simulink model "mte484lab3partc2"  (R2024a)
settings: Solver=VariableStepAuto  StartTime=0.0  StopTime=60.0  MaxStep=0.001  RelTol=1e-3
values from neighbouring files (symbols this model uses):
  C2den = [1 Pd(2) 0]    [mte484lab3partcsetup.m]
  C2num = [-7 -2.45]    [mte484lab3partasetup.m]    (also in mte484lab3partcsetup.m = -Pd(3:5)/g)
  Cden = [1 pc]    [mte484lab3partcsetup.m]
  Cnum = -k*[1 zc]    [mte484lab3partcsetup.m]
  K1 = -1.883    [mte484lab3partcsetup.m]
  K2 = 0.0609    [mte484lab3parta.m]    (also in mte484lab3partasetup.m; mte484lab3partcsetup.m)
  K3 = -4.526    [mte484lab3parta.m]    (also in mte484lab3partasetup.m; mte484lab3partcsetup.m)
  sat = 0.7    [mte484lab3parta.m]    (also in mte484lab3partasetup.m; mte484lab3partcsetup.m)
  tau = 0.0216    [mte484lab3partcsetup.m]
  Ts = 0.001    [mte484lab3parta.m]    (also in mte484lab3partasetup.m; mte484lab3partbsetup.m; mte484lab3partcsetup.m)
undefined symbols (not defined in the file or in its folder): D2den, D2num, Dden, Dnum
settings Model: Creator=christopherkoo  LastModifiedBy=christopherkoo

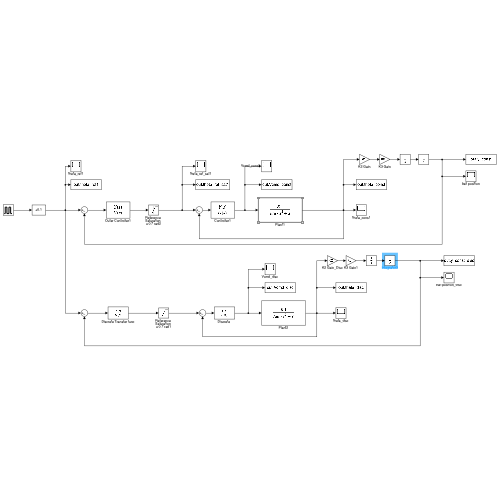
[thumbnail: Simulink's stored preview of the top-level diagram]
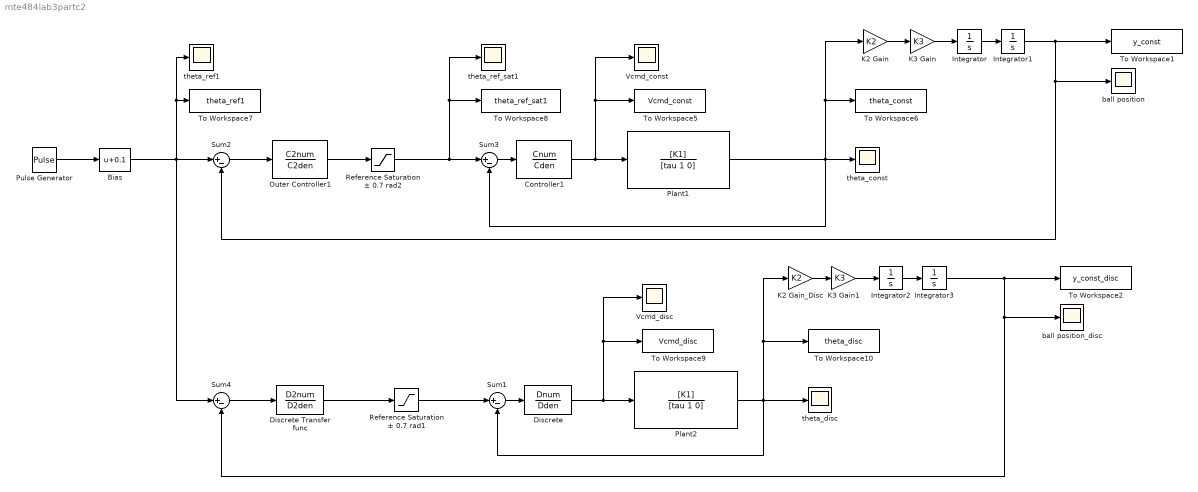
== system mte484lab3partc2 ==
  Bias : Bias  Bias=0.1  SaturateOnIntegerOverflow=off
  Controller1 : TransferFcn  Numerator=Cnum  Denominator=Cden
  "Discrete " : DiscreteTransferFcn  Numerator=Dnum  Denominator=Dden  SampleTime=Ts
  Discrete Transfer func : DiscreteTransferFcn  Numerator=D2num  Denominator=D2den  SampleTime=Ts
  Integrator : Integrator
  Integrator1 : Integrator  InitialCondition=0.1
  Integrator2 : Integrator
  Integrator3 : Integrator  InitialCondition=0.1
  K2 Gain : Gain  Gain=K2
  K2 Gain_Disc : Gain  Gain=K2
  K3 Gain : Gain  Gain=K3
  K3 Gain1 : Gain  Gain=K3
  Outer Controller1 : TransferFcn  Numerator=C2num  Denominator=C2den
  Plant1 : TransferFcn  Numerator=[K1]  Denominator=[tau 1 0]
  Plant2 : TransferFcn  Numerator=[K1]  Denominator=[tau 1 0]
  Pulse Generator : DiscretePulseGenerator  PulseType=Time based  Amplitude=0.15  Period=20  PulseWidth=50
  Reference Saturation ± 0.7 rad1 : Saturate  UpperLimit=sat  LowerLimit=-sat
  Reference Saturation ± 0.7 rad2 : Saturate  UpperLimit=sat  LowerLimit=-sat
  Sum{1..4} (4 alike) : Sum  Inputs=|+-
  To Workspace1 : ToWorkspace  VariableName=y_const  SaveFormat=Timeseries  SampleTime=-1
  To Workspace10 : ToWorkspace  VariableName=theta_disc  SaveFormat=Timeseries  SampleTime=-1
  To Workspace2 : ToWorkspace  VariableName=y_const_disc  SaveFormat=Timeseries  SampleTime=-1
  To Workspace5 : ToWorkspace  VariableName=Vcmd_const  SaveFormat=Timeseries  SampleTime=-1
  To Workspace6 : ToWorkspace  VariableName=theta_const  SaveFormat=Timeseries  SampleTime=-1
  To Workspace7 : ToWorkspace  VariableName=theta_ref1  SaveFormat=Timeseries  SampleTime=-1
  To Workspace8 : ToWorkspace  VariableName=theta_ref_sat1  SaveFormat=Timeseries  SampleTime=-1
  To Workspace9 : ToWorkspace  VariableName=Vcmd_disc  SaveFormat=Timeseries  SampleTime=-1
  Vcmd_const : Scope
  Vcmd_disc : Scope
  ball position : Scope
  ball position_disc : Scope
  theta_const : Scope
  theta_disc : Scope
  theta_ref1 : Scope
  theta_ref_sat1 : Scope
  wires:
  Bias/1 -> Sum4/1, Sum2/1, theta_ref1/1, To Workspace7/1
  Controller1/1 -> Plant1/1, Vcmd_const/1, To Workspace5/1
  Sum1/1 -> "Discrete "/1
  Sum3/1 -> Controller1/1
  Plant2/1 -> K2 Gain_Disc/1, To Workspace10/1, theta_disc/1, Sum1/2
  "Discrete "/1 -> Plant2/1, Vcmd_disc/1, To Workspace9/1
  Reference Saturation ± 0.7 rad2/1 -> To Workspace8/1, theta_ref_sat1/1, Sum3/1
  Outer Controller1/1 -> Reference Saturation ± 0.7 rad2/1
  Sum2/1 -> Outer Controller1/1
  Plant1/1 -> Sum3/2, K2 Gain/1, To Workspace6/1, theta_const/1
  K2 Gain/1 -> K3 Gain/1
  Integrator1/1 -> To Workspace1/1, ball position/1, Sum2/2
  Pulse Generator/1 -> Bias/1
  Reference Saturation ± 0.7 rad1/1 -> Sum1/1
  Discrete Transfer func/1 -> Reference Saturation ± 0.7 rad1/1
  Sum4/1 -> Discrete Transfer func/1
  Integrator3/1 -> To Workspace2/1, Sum4/2, ball position_disc/1
  K3 Gain/1 -> Integrator/1
  Integrator/1 -> Integrator1/1
  K2 Gain_Disc/1 -> K3 Gain1/1
  K3 Gain1/1 -> Integrator2/1
  Integrator2/1 -> Integrator3/1
